simulink model "basebot_model_sampling"  (R2026a)
settings: Solver=VariableStepAuto  MaxStep=1e-4
values from neighbouring files (symbols this model uses):
  den = conv([L R], [J D]) + [0 0 K^2]    [compareRobot.m]    (also in driveModel.m; driveSquare.m; piDesign.mat = [3.18211752541e-08 2.39694947115e-05 7.04575028668e-05]; samplingModel.m)
  gear = 9.6    [buildExercise1Models.m]    (also in compareRobot.m; driveModel.m; driveSquare.m; finalProjectModel.m)
  Kp = runs{n,2}    [compareRobot.m]    (also in driveSquare.m = 0.02; piDesign.m = 0.13; piDesign.mat = 0.13; samplingModel.m = 0.05)
  num = K    [compareRobot.m]    (also in driveModel.m; driveSquare.m; piDesign.mat = 0.00812424172394; samplingModel.m)
  r = 0.0315    [compareRobot.m]    (also in driveModel.m; driveSquare.m; finalProjectModel.m; samplingModel.m)
  T = 0.010    (= 0.01)    [compareRobot.m]    (also in piDesign.mat; samplingModel.m; transferFunction.m)
  Ts = 0.001;'    [buildExercise1Models.m]    (also in compareRobot.m = round(median(diff(t)), 4); driveModel.m = 0.001; driveSquare.m = 0.001; finalProjectModel.m = 0.001)
  Vmax = 9    [compareRobot.m]    (also in driveModel.m; driveSquare.m; finalProjectModel.m; piDesign.m = 8)
settings Model: Creator=bidaze  LastModifiedBy=bidaze

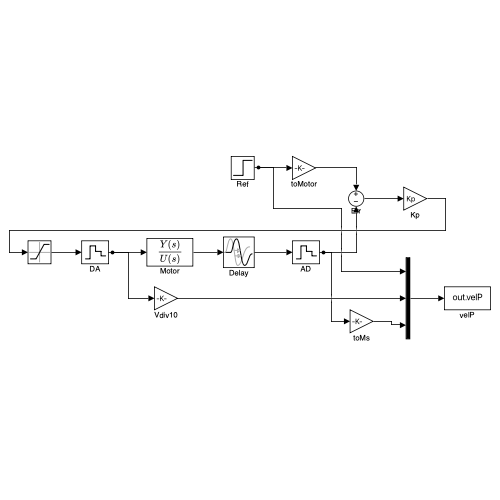
[thumbnail: Simulink's stored preview of the top-level diagram]
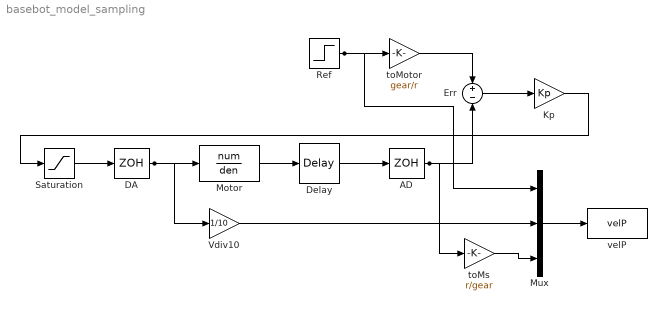
== system basebot_model_sampling ==
  AD : ZeroOrderHold  SampleTime=Ts
  DA : ZeroOrderHold  SampleTime=Ts
  Delay : TransportDelay  DelayTime=T
  Err : Sum  Inputs=+-
  Kp : Gain  Gain=Kp
  Motor : TransferFcn  Numerator=num  Denominator=den
  Mux : Mux  Inputs=3
  Ref : Step  Time=0.2  FinalValue=0.1  SampleTime=0
  Saturation : Saturate  UpperLimit=Vmax  LowerLimit=-Vmax
  Vdiv10 : Gain  Gain=1/10
  toMotor : Gain  Gain=gear/r
  toMs : Gain  Gain=r/gear
  velP : ToWorkspace  VariableName=velP  SaveFormat=Timeseries  SampleTime=-1
  wires:
  toMs/1 -> Mux/3
  Err/1 -> Kp/1
  Kp/1 -> Saturation/1
  AD/1 -> toMs/1, Err/2
  toMotor/1 -> Err/1
  Delay/1 -> AD/1
  Mux/1 -> velP/1
  Motor/1 -> Delay/1
  Saturation/1 -> DA/1
  Vdiv10/1 -> Mux/2
  DA/1 -> Vdiv10/1, Motor/1
  Ref/1 -> toMotor/1, Mux/1
